simulink model "implfb_can_pack"  (R2026b)
settings: Solver=VariableStepAuto
undefined symbols (not defined in the file or in its folder): Ts
libraries: svdutilitieslib x1, simulink x1
settings Model: Creator=aomar  LastModifiedBy=aomar

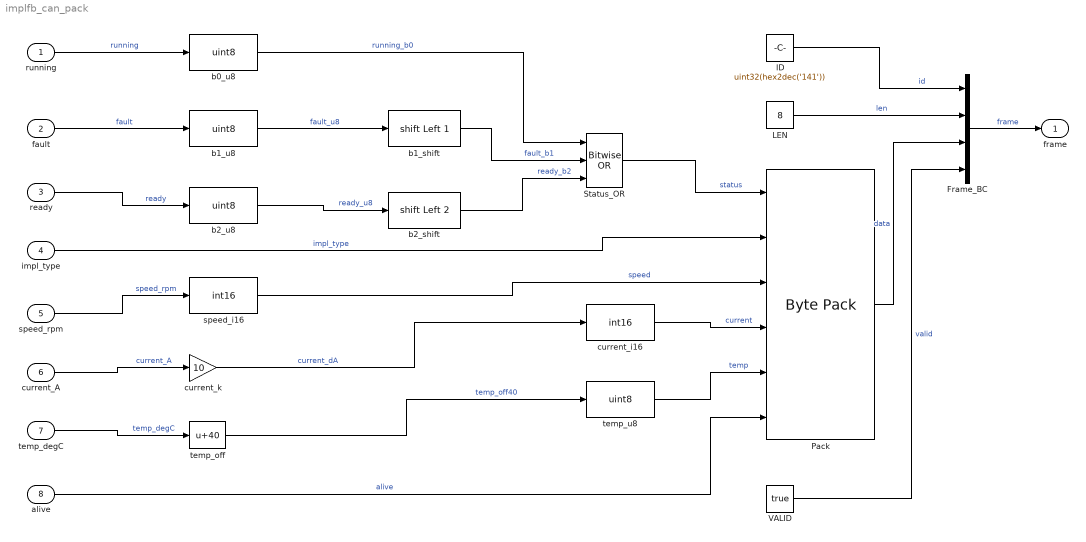
== system implfb_can_pack ==
  running : Inport  OutDataTypeStr=boolean  PortDimensions=1  SampleTime=Ts.can_slow
  fault : Inport  Port=2  OutDataTypeStr=boolean  PortDimensions=1  SampleTime=Ts.can_slow
  ready : Inport  Port=3  OutDataTypeStr=boolean  PortDimensions=1  SampleTime=Ts.can_slow
  impl_type : Inport  Port=4  OutDataTypeStr=uint8  PortDimensions=1  SampleTime=Ts.can_slow
  speed_rpm : Inport  Port=5  OutDataTypeStr=single  PortDimensions=1  SampleTime=Ts.can_slow
  current_A : Inport  Port=6  OutDataTypeStr=single  PortDimensions=1  SampleTime=Ts.can_slow
  temp_degC : Inport  Port=7  OutDataTypeStr=single  PortDimensions=1  SampleTime=Ts.can_slow
  alive : Inport  Port=8  OutDataTypeStr=uint8  PortDimensions=1  SampleTime=Ts.can_slow
  Frame_BC : BusCreator  Inputs=4  OutDataTypeStr=Bus: Bus_CanFrame8  NonVirtualBus=on
      settings: InheritFromInputs=off
  ID : Constant  Value=uint32(hex2dec('141'))  OutDataTypeStr=uint32  SampleTime=Ts.can_slow
  LEN : Constant  Value=8  OutDataTypeStr=uint8  SampleTime=Ts.can_slow
  Pack : svdutilitieslib/Byte Pack  maskPackedDataType=uint8  datatypes={'uint8','uint8','int16','int16','uint8','uint8'}  byteAlign=1  blockPlatform=arduinoert
      settings: LibrarySourceBlock=mcblib/Signal Management/Byte Pack
  Status_OR : simulink/Logic and Bit Operations/Bitwise Operator  logicop=OR  UseBitMask=off  NumInputPorts=3  BitMask=bin2dec('11011001')  BitMaskRealWorld=Stored Integer
  VALID : Constant  Value=true  OutDataTypeStr=boolean  SampleTime=Ts.can_slow
  b0_u8 : DataTypeConversion  OutDataTypeStr=uint8  RndMeth=Nearest
  b1_shift : ArithShift  BitShiftNumber=1  BitShiftDirection=Left
  b1_u8 : DataTypeConversion  OutDataTypeStr=uint8  RndMeth=Nearest
  b2_shift : ArithShift  BitShiftNumber=2  BitShiftDirection=Left
  b2_u8 : DataTypeConversion  OutDataTypeStr=uint8  RndMeth=Nearest
  current_i16 : DataTypeConversion  OutDataTypeStr=int16  RndMeth=Nearest
  current_k : Gain  Gain=10
  speed_i16 : DataTypeConversion  OutDataTypeStr=int16  RndMeth=Nearest
  temp_off : Bias  Bias=40  SaturateOnIntegerOverflow=off
  temp_u8 : DataTypeConversion  OutDataTypeStr=uint8  RndMeth=Nearest
  frame : Outport  OutDataTypeStr=Bus: Bus_CanFrame8
  wires:
  running/1 -> b0_u8/1  "running"
  fault/1 -> b1_u8/1  "fault"
  ready/1 -> b2_u8/1  "ready"
  impl_type/1 -> Pack/2  "impl_type"
  speed_rpm/1 -> speed_i16/1  "speed_rpm"
  current_A/1 -> current_k/1  "current_A"
  temp_degC/1 -> temp_off/1  "temp_degC"
  alive/1 -> Pack/6  "alive"
  current_k/1 -> current_i16/1  "current_dA"
  temp_off/1 -> temp_u8/1  "temp_off40"
  b0_u8/1 -> Status_OR/1  "running_b0"
  b1_u8/1 -> b1_shift/1  "fault_u8"
  b2_u8/1 -> b2_shift/1  "ready_u8"
  speed_i16/1 -> Pack/3  "speed"
  b1_shift/1 -> Status_OR/2  "fault_b1"
  b2_shift/1 -> Status_OR/3  "ready_b2"
  Status_OR/1 -> Pack/1  "status"
  current_i16/1 -> Pack/4  "current"
  temp_u8/1 -> Pack/5  "temp"
  ID/1 -> Frame_BC/1  "id"
  LEN/1 -> Frame_BC/2  "len"
  VALID/1 -> Frame_BC/4  "valid"
  Pack/1 -> Frame_BC/3  "data"
  Frame_BC/1 -> frame/1  "frame"
